simulink model "quad_full_6dof"  (R2026a)
settings: Solver=ode4  StopTime=sim_stop_time  FixedStep=sim_dt
PreLoadFcn:
  | quad_params
values from neighbouring files (symbols this model uses):
  a_max = 2.0    (= 2)    [all_parameters.m]    (also in combined_params_all.m; quad_params.m)
  att_lim = 25*pi/180    (= 0.436332312999)    [all_parameters.m]    (also in combined_params_all.m; quad_params.m)
  g = 9.81    [all_parameters.m]    (also in combined_params_all.m; fdi_ftc_test_suite.m = [g 'end']; ftc_design_delta.m = P.g; quad_params.m)
  Jxx = 54737.66e-9    (= 5.473766e-05)    [all_parameters.m]    (also in combined_params_all.m; quad_params.m)
  Jyy = 53435.96e-9    (= 5.343596e-05)    [all_parameters.m]    (also in combined_params_all.m; quad_params.m)
  Jzz = 98934.3e-9    (= 9.89343e-05)    [all_parameters.m]    (also in combined_params_all.m; quad_params.m)
  Kd_p = 12*Jyy    (= 0.00064123152)    [all_parameters.m]    (also in combined_params_all.m; quad_params.m)
  Kd_pos = 1.8    [all_parameters.m]    (also in combined_params_all.m; quad_params.m)
  Kd_r = 12*Jxx    (= 0.00065685192)    [all_parameters.m]    (also in combined_params_all.m; quad_params.m)
  Kd_y = 2.5*Jzz    (= 0.00024733575)    [all_parameters.m]    (also in combined_params_all.m; quad_params.m)
  kf = 5e-8    (= 5e-08)    [all_parameters.m]    (also in combined_params_all.m; fdi_ftc_test_suite.m = P.kf; ftc_design_delta.m = P.kf; quad_params.m)
  Kp_p = 60*Jyy    (= 0.0032061576)    [all_parameters.m]    (also in combined_params_all.m; quad_params.m)
  Kp_pos = 1.2    [all_parameters.m]    (also in combined_params_all.m; quad_params.m)
  Kp_r = 60*Jxx    (= 0.0032842596)    [all_parameters.m]    (also in combined_params_all.m; quad_params.m)
  Kp_y = 3*Jzz    (= 0.0002968029)    [all_parameters.m]    (also in combined_params_all.m; quad_params.m)
  kt = 0.025*kf    (= 1.25e-09)    [all_parameters.m]    (also in combined_params_all.m; fdi_ftc_test_suite.m = P.kt; ftc_design_delta.m = P.kt; quad_params.m)
  l = 54.33e-3    (= 0.05433)    [all_parameters.m]    (also in combined_params_all.m; fdi_ftc_test_suite.m = P.l; ftc_design_delta.m = P.l; quad_params.m)
  m = (75 + 45.7)/1000    (= 0.1207)    [all_parameters.m]    (also in combined_params_all.m; fdi_ftc_test_suite.m = P.m; ftc_design_delta.m = P.m; quad_params.m)
  om0 = [0; 0; 0]    [all_parameters.m]    (also in combined_params_all.m; quad_params.m)
  p0 = [0; 0; 0]    [all_parameters.m]    (also in combined_params_all.m; quad_params.m)
  psi_step_time = 7.0    (= 7)    [all_parameters.m]    (also in combined_params_all.m; quad_params.m)
  q0 = [1; 0; 0; 0]    [all_parameters.m]    (also in combined_params_all.m; quad_params.m)
  tau = 0.02    [all_parameters.m]    (also in combined_params_all.m; fdi_ftc_test_suite.m = P.tau; ftc_design_delta.m = P.tau; quad_params.m)
  v0 = [0; 0; 0]    [all_parameters.m]    (also in combined_params_all.m; quad_params.m)
  w_max = 2.5*sqrt(m*g/(4*kf))    [all_parameters.m]    (also in combined_params_all.m; quad_params.m)
settings Model: Creator=UCT  LastModifiedBy=UCT

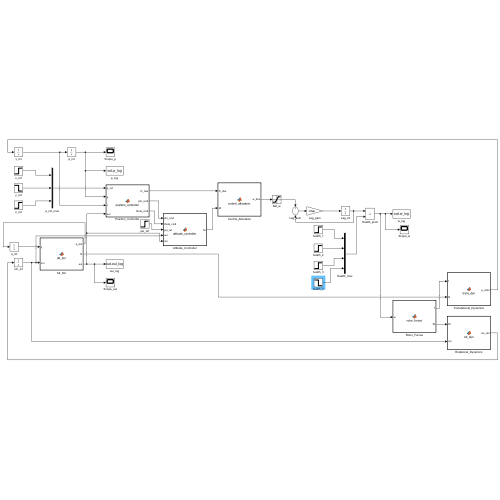
[thumbnail: Simulink's stored preview of the top-level diagram]
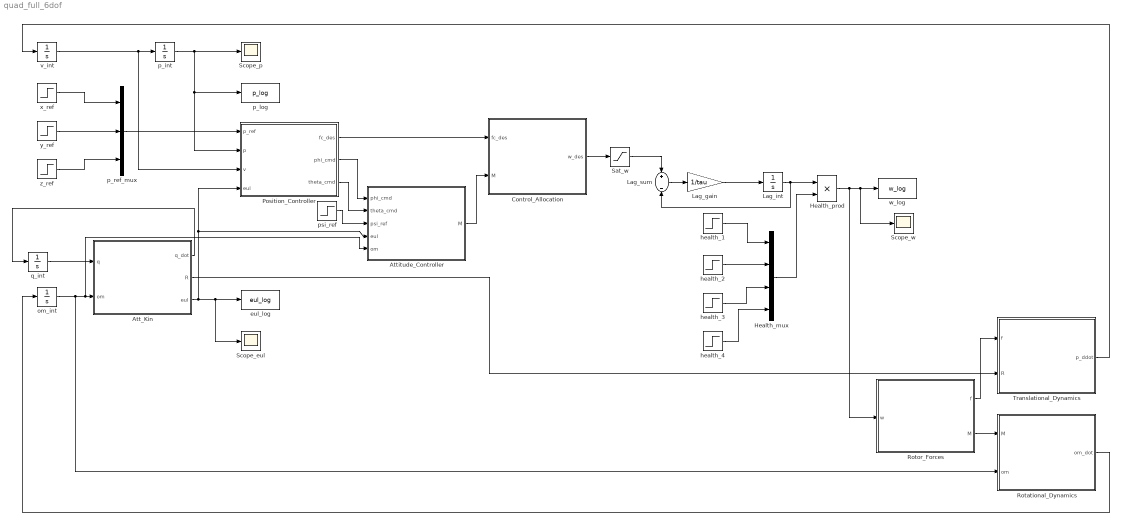
== system quad_full_6dof ==
  Att_Kin : MATLAB Function  TreatAsAtomicUnit=on
  Attitude_Controller : MATLAB Function  TreatAsAtomicUnit=on
  Control_Allocation : MATLAB Function  TreatAsAtomicUnit=on
  Health_mux : Mux
  Health_prod : Product
  Lag_gain : Gain  Gain=1/tau
  Lag_int : Integrator  InitialCondition=sqrt(m*g/(4*kf))*ones(4,1)
  Lag_sum : Sum  Inputs=+-
  Position_Controller : MATLAB Function  TreatAsAtomicUnit=on
  Rotational_Dynamics : MATLAB Function  TreatAsAtomicUnit=on
  Rotor_Forces : MATLAB Function  TreatAsAtomicUnit=on
  Sat_w : Saturate  UpperLimit=w_max  LowerLimit=0
  Scope_eul : Scope
      settings: ActiveDisplayYMinimum=-4.7929691132816243  ActiveDisplayYMaximum=4.7594431043530188
  Scope_p : Scope
  Scope_w : Scope
  Translational_Dynamics : MATLAB Function  TreatAsAtomicUnit=on
  eul_log : ToWorkspace  VariableName=eul_log  SaveFormat=Timeseries  SampleTime=-1
  health_1 : Step  Time=15  InitialValue=1  SampleTime=0
  health_2 : Step  Time=15  InitialValue=1  SampleTime=0
  health_3 : Step  Time=15  InitialValue=1  SampleTime=0
  health_4 : Step  Time=14  InitialValue=1  FinalValue=0  SampleTime=0
  om_int : Integrator  InitialCondition=om0
  p_int : Integrator  InitialCondition=p0
  p_log : ToWorkspace  VariableName=p_log  SaveFormat=Timeseries  SampleTime=-1
  p_ref_mux : Mux  Inputs=3
  psi_ref : Step  Time=psi_step_time  FinalValue=psi_step_value  SampleTime=0
  q_int : Integrator  InitialCondition=q0
  v_int : Integrator  InitialCondition=v0
  w_log : ToWorkspace  VariableName=w_log  SaveFormat=Timeseries  SampleTime=-1
  x_ref : Step  Time=9  FinalValue=3  SampleTime=0
  y_ref : Step  Time=6  FinalValue=-5  SampleTime=0
  z_ref : Step  Time=0.5  FinalValue=5  SampleTime=0
  wires:
  p_int/1 -> Position_Controller/2(p), p_log/1, Scope_p/1
  om_int/1 -> Attitude_Controller/5(om), Att_Kin/2(om), Rotational_Dynamics/2(om)
  psi_ref/1 -> Attitude_Controller/3(psi_ref)
  v_int/1 -> Position_Controller/3(v), p_int/1
  x_ref/1 -> p_ref_mux/1
  y_ref/1 -> p_ref_mux/2
  p_ref_mux/1 -> Position_Controller/1(p_ref)
  z_ref/1 -> p_ref_mux/3
  q_int/1 -> Att_Kin/1(q)
  Att_Kin/1(q_dot) -> q_int/1
  Att_Kin/2(R) -> Translational_Dynamics/2(R)
  Att_Kin/3(eul) -> eul_log/1, Scope_eul/1, Attitude_Controller/4(eul), Position_Controller/4(eul)
  Position_Controller/1(fc_des) -> Control_Allocation/1(fc_des)
  Position_Controller/2(phi_cmd) -> Attitude_Controller/1(phi_cmd)
  Position_Controller/3(theta_cmd) -> Attitude_Controller/2(theta_cmd)
  Health_prod/1 -> w_log/1, Scope_w/1, Rotor_Forces/1(w)
  Lag_int/1 -> Health_prod/1, Lag_sum/2
  health_1/1 -> Health_mux/1
  Attitude_Controller/1(M) -> Control_Allocation/2(M)
  Control_Allocation/1(w_des) -> Sat_w/1
  Sat_w/1 -> Lag_sum/1
  Lag_sum/1 -> Lag_gain/1
  Lag_gain/1 -> Lag_int/1
  health_2/1 -> Health_mux/2
  Health_mux/1 -> Health_prod/2
  health_3/1 -> Health_mux/3
  health_4/1 -> Health_mux/4
  Rotational_Dynamics/1(om_dot) -> om_int/1
  Rotor_Forces/1(f) -> Translational_Dynamics/1(f)
  Rotor_Forces/2(M) -> Rotational_Dynamics/1(M)
  Translational_Dynamics/1(p_ddot) -> v_int/1

== matlab function quad_full_6dof/Attitude_Controller ==
  data: phi_cmd input; M output; theta_cmd input; psi_ref input; eul input; om input; Kp_r parameter; Kd_r parameter; Kp_p parameter; Kd_p parameter; Kp_y parameter; Kd_y parameter
function M = attitude_controller(phi_cmd, theta_cmd, psi_ref, eul, om, Kp_r, Kd_r, Kp_p, Kd_p, Kp_y, Kd_y)
e = eul(:); o = om(:);
e_psi = atan2(sin(psi_ref - e(3)), cos(psi_ref - e(3)));   % wrapped yaw error
Mx = Kp_r*(phi_cmd   - e(1)) - Kd_r*o(1);
My = Kp_p*(theta_cmd - e(2)) - Kd_p*o(2);
Mz = Kp_y*e_psi           - Kd_y*o(3);
M = [Mx; My; Mz];
end

% checks the command pitch, roll and yaw angles respective to where they
% have to be and then outputs the torque required to correct the error is
% there is

== matlab function quad_full_6dof/Position_Controller ==
  data: p_ref input; fc_des output; p input; v input; eul input; phi_cmd output; theta_cmd output; Kp_pos parameter; Kd_pos parameter; a_max parameter; att_lim parameter; g parameter; m parameter
function [fc_des, phi_cmd, theta_cmd] = position_controller(p_ref, p, v, eul, Kp_pos, Kd_pos, a_max, att_lim, g, m)

% check where the quadcopter is with respect to where it has to be and then.
% outputs the desired thrust and pitch and roll angles 

pr = p_ref(:); pp = p(:); vv = v(:); e = eul(:);
phi = e(1); theta = e(2); psi = e(3);
a = Kp_pos*(pr - pp) - Kd_pos*vv;
a = max(min(a, a_max), -a_max);
lim = att_lim;

% rotate desired x/y acceleration into the yaw-aligned frame, small-angle map
theta_cmd = max(min((a(1)*cos(psi) + a(2)*sin(psi))/g, lim), -lim);
phi_cmd   = max(min((a(1)*sin(psi) - a(2)*cos(psi))/g, lim), -lim);

% collective thrust with tilt compensation
fc_des = m*(g + a(3))/max(cos(phi)*cos(theta), 0.5);
end

== matlab function quad_full_6dof/Control_Allocation ==
  data: fc_des input; w_des output; M input; kf parameter; kt parameter; l parameter
function w_des = control_allocation(fc_des, M, kf, kt, l)
Mv = M(:);
Mx = Mv(1); My = Mv(2); Mz = Mv(3);
w1sq = fc_des/(4*kf) - My/(2*l*kf) + Mz/(4*kt);
w2sq = fc_des/(4*kf) - Mx/(2*l*kf) - Mz/(4*kt);
w3sq = fc_des/(4*kf) + My/(2*l*kf) + Mz/(4*kt);
w4sq = fc_des/(4*kf) + Mx/(2*l*kf) - Mz/(4*kt);
w_des = sqrt(max([w1sq; w2sq; w3sq; w4sq], 0));
end

== matlab function quad_full_6dof/Rotor_Forces ==
  data: w input; f output; M output; kf parameter; kt parameter; l parameter
function [f, M] = rotor_forces(w, kf, kt, l)
w2 = w(:).^2;
f = kf*sum(w2);
M = [l*kf*(w2(4) - w2(2)); ...
     l*kf*(w2(3) - w2(1)); ...
     kt*(w2(1) - w2(2) + w2(3) - w2(4))];
end

%It takes the four rotor speeds and returns the total thrust and the three body torques that those speeds produce.

== matlab function quad_full_6dof/Rotational_Dynamics ==
  data: M input; om_dot output; om input; Jxx parameter; Jyy parameter; Jzz parameter
function om_dot = rot_dyn(M, om, Jxx, Jyy, Jzz)
% J*om_dot + om x (J*om) = M   (J diagonal)
Mv = M(:); o = om(:);
Jv = [Jxx; Jyy; Jzz];
om_dot = (Mv - cross(o, Jv.*o))./Jv;
end

== matlab function quad_full_6dof/Att_Kin ==
  data: q input; q_dot output; om input; R output; eul output
function [q_dot, R, eul] = att_kin(q, om)
qv = q(:); o = om(:);
qn = qv/norm(qv); %normalising  
qa = qn(1); q1 = qn(2); q2 = qn(3); q3 = qn(4);
p = o(1); qq = o(2); r = o(3);

%quaternion multiplication 
q_dot = 0.5*[-q1*p - q2*qq - q3*r; ...
              qa*p + q2*r - q3*qq; ...
              qa*qq - q1*r + q3*p; ...
              qa*r + q1*qq - q2*p];
%quaternion to rotational matrix 
R = [1-2*(q2^2+q3^2), 2*(q1*q2-qa*q3),   2*(q1*q3+qa*q2); ...
     2*(q1*q2+qa*q3), 1-2*(q1^2+q3^2),   2*(q2*q3-qa*q1); ...
     2*(q1*q3-qa*q2), 2*(q2*q3+qa*q1),   1-2*(q1^2+q2^2)];

%quaternion to euler 
phi   = atan2(2*(qa*q1+q2*q3), 1-2*(q1^2+q2^2));
theta = asin(max(-1, min(1, 2*(qa*q2-q3*q1))));
psi   = atan2(2*(qa*q3+q1*q2), 1-2*(q2^2+q3^2));
eul = [phi; theta; psi];
end

== matlab function quad_full_6dof/Translational_Dynamics ==
  data: f input; p_ddot output; R input; m parameter; g parameter
function p_ddot = trans_dyn(f, R, m, g)
% m*p_ddot = WR_B*[0;0;f] + [0;0;-m*g]
p_ddot = (R*[0; 0; f] + [0; 0; -m*g])/m;
end
